simulink model "Prj1CDig_ZOH"  (R2026b)
settings: Solver=ode23s  StopTime=3600  RelTol=1e-8  EnableMultiTasking=on
undefined symbols (not defined in the file): Am, AmpW0, Bm, DiscIntNeverNeededParam, KI, KP, Kp, PO, Sat, Ta, Td, Tp1, Tp2, Ts, w0
settings Model: Creator=Adolfo  LastModifiedBy=Santana
settings SolverCC: MaxConsecutiveMinStep=5  ZeroCrossControl=DisableAll
settings DataIOCC: LimitDataPoints=on  MaxDataPoints=25000  ReturnWorkspaceOutputs=off  SaveFormat=Array  SignalLoggingSaveFormat=ModelDataLogs
settings OptimizationCC: BlockReduction=off  BooleanDataType=off  LifeSpan=inf  MemsetInitFltsAndDblsToZero=off  ReuseModelBlockBuffer=off
settings DebuggingCC: ArithmeticOperatorsInVariantConditions=warning  FcnCallInpInsideContextMsg=warning  MergeDetectMultiDrivingBlocksExec=none  MultiTaskCondExecSysMsg=none  MultiTaskDSMMsg=warning  SFExecutionAtInitializationDiag=none  SFNoUnconditionalDefaultTransitionDiag=warning  SFUnexpectedBacktrackingDiag=warning  SaveWithParameterizedLinksMsg=none  SignalResolutionControl=TryResolveAllWithWarning  StateNameClashWarn=warning  UnderspecifiedInitializationDetection=Classic
settings HardwareCC: ProdEndianess=Unspecified  ProdHWDeviceType=32-bit Generic  ProdIntDivRoundTo=Undefined  ProdLargestAtomicFloat=None  TargetUnknown=on
settings ModelReferenceCC: PropagateSignalLabelsOutOfModel=off
settings SFSimCC: CustomCodeUndefinedFunction=UseInterfaceOnly  SimUseLocalCustomCode=off
settings RTWCC: RTWUseLocalCustomCode=off
settings CodeAppCC: StateflowObjectComments=on
settings GRTTargetCC: CombineOutputUpdateFcns=off  GRTInterface=on  TargetFcnLib=ansi_tfl_tmw.mat  TargetLangStandard=C89/C90 (ANSI)
settings ConfigComp: CovSaveCumulativeToWorkspaceVar=on  CovSaveSingleToWorkspaceVar=on

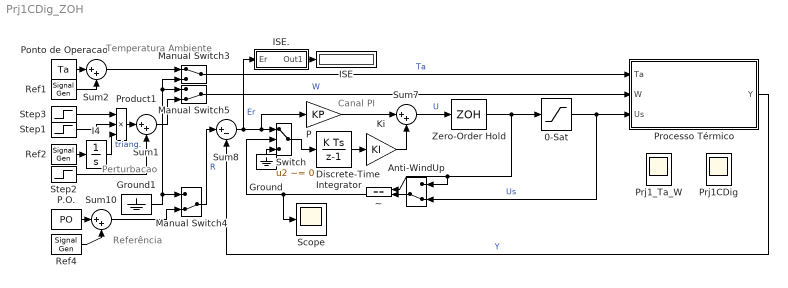
== system Prj1CDig_ZOH ==
  note: Referência
  note: Perturbacao
  note: Canal PI
  note: Temperatura Ambiente
  0-Sat : Saturate  UpperLimit=Sat  LowerLimit=0
  Anti-WindUp : ManualSwitch  CurrentSetting=0
  Discrete-Time Integrator : DiscreteIntegrator  SampleTime=Ts  ICPrevOutput=DiscIntNeverNeededParam  ICPrevScaledInput=DiscIntNeverNeededParam
  Ground : Ground
  Ground1 : Ground
  I4 : Integrator
  ISE : Display
  ISE. : Subsystem
  Ki : Gain  Gain=KI
  Manual Switch3 : ManualSwitch
  Manual Switch4 : ManualSwitch  CurrentSetting=0
  Manual Switch5 : ManualSwitch  CurrentSetting=0
  P : Gain  Gain=KP
  P.O. : Constant  Value=PO
  Ponto de Operacao : Constant  Value=Ta
  Prj1CDig : Scope
      settings: IsFloating=on  Floating=on  TimeSpan=3600  ActiveDisplayYMinimum=-200  ActiveDisplayYMaximum=1400  DataLoggingVariableName=ScopeData2
  Prj1_Ta_W : Scope
      settings: IsFloating=on  Floating=on  TimeSpan=3600  ActiveDisplayYMinimum=-25  ActiveDisplayYMaximum=35
  Processo Térmico : Subsystem
  Product1 : Product  Inputs=3  RndMeth=Zero
  Ref1 : SignalGenerator  Amplitude=2  Frequency=1/3600/24
  Ref2 : SignalGenerator  WaveForm=square  Amplitude=AmpW0  Frequency=w0  Units=rad/sec
  Ref4 : SignalGenerator  WaveForm=square  Amplitude=5  Frequency=.00125
  Scope : Scope
      settings: ActiveDisplayYMinimum=-0.125  ActiveDisplayYMaximum=1.125
  Step1 : Step  Time=3000  InitialValue=-20  FinalValue=0  SampleTime=0
  Step2 : Step  Time=1000  FinalValue=-20  SampleTime=0
  Step3 : Step  Time=1800  SampleTime=0
  Sum{1..2,7,10} (4 alike) : Sum  Inputs=|++
  Sum8 : Sum  Inputs=|+-
  Switch : Switch  Criteria=u2 ~= 0  Threshold=1  SaturateOnIntegerOverflow=off  InputSameDT=off
  Zero-Order Hold : ZeroOrderHold  SampleTime=Ts
  ~ : RelationalOperator  Operator===  OutDataTypeStr=boolean  InputSameDT=off
  wires:
  Sum8/1 -> P/1, Switch/1, ISE./1(Er)  "Er"
  P/1 -> Sum7/1
  Manual Switch5/1 -> Processo Térmico/2(W)  "W"
  Manual Switch3/1 -> Processo Térmico/1(Ta)  "Ta"
  Ground1/1 -> Manual Switch4/1, Manual Switch5/1, Manual Switch3/2
  Manual Switch4/1 -> Sum8/1  "R"
  Sum1/1 -> Manual Switch5/2
  Sum2/1 -> Manual Switch3/1
  Sum10/1 -> Manual Switch4/2
  Step2/1 -> Sum1/2
  Product1/1 -> Sum1/1
  Processo Térmico/1(Y) -> Sum8/2  "Y"
  Sum7/1 -> Zero-Order Hold/1  "U"
  Step1/1 -> Product1/2
  Step3/1 -> Product1/1
  Ref2/1 -> I4/1
  P.O./1 -> Sum10/1
  Ref4/1 -> Sum10/2
  ISE./1(Out1) -> ISE/1
  I4/1 -> Product1/3  "triang."
  Ki/1 -> Sum7/2
  0-Sat/1 -> Anti-WindUp/2, Processo Térmico/3(Us)  "Us"
  ~/1 -> Scope/1, Switch/2
  Anti-WindUp/1 -> ~/2
  Ground/1 -> Switch/3
  Discrete-Time Integrator/1 -> Ki/1
  Switch/1 -> Discrete-Time Integrator/1
  Ref1/1 -> Sum2/2
  Ponto de Operacao/1 -> Sum2/1
  Zero-Order Hold/1 -> 0-Sat/1, Anti-WindUp/1, ~/1

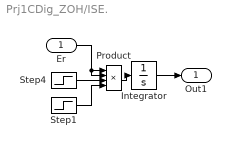
== system Prj1CDig_ZOH/ISE. ==
  Er : Inport
  Integrator : Integrator
  Product : Product  Inputs=4  RndMeth=Zero
  Step1 : Step  Time=3000  InitialValue=1  FinalValue=0  SampleTime=0
  Step4 : Step  Time=2100  SampleTime=0
  Out1 : Outport
  wires:
  Integrator/1 -> Out1/1
  Product/1 -> Integrator/1
  Step4/1 -> Product/3
  Er/1 -> Product/2, Product/1
  Step1/1 -> Product/4

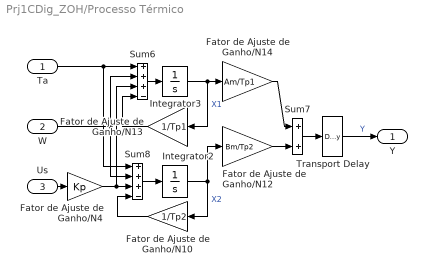
== system Prj1CDig_ZOH/Processo Térmico ==
  Ta : Inport
  W : Inport  Port=2
  Us : Inport  Port=3
  Fator de Ajuste de Ganho/N10 : Gain  Gain=1/Tp2  SaturateOnIntegerOverflow=on  OutDataTypeStr=Inherit: Same as input  ParamDataTypeStr=Inherit: Same as input
  Fator de Ajuste de Ganho/N12 : Gain  Gain=Bm/Tp2  SaturateOnIntegerOverflow=on  OutDataTypeStr=Inherit: Same as input  ParamDataTypeStr=Inherit: Same as input
  Fator de Ajuste de Ganho/N13 : Gain  Gain=1/Tp1  SaturateOnIntegerOverflow=on  OutDataTypeStr=Inherit: Same as input  ParamDataTypeStr=Inherit: Same as input
  Fator de Ajuste de Ganho/N14 : Gain  Gain=Am/Tp1  SaturateOnIntegerOverflow=on  OutDataTypeStr=Inherit: Same as input  ParamDataTypeStr=Inherit: Same as input
  Fator de Ajuste de Ganho/N4 : Gain  Gain=Kp  SaturateOnIntegerOverflow=on  OutDataTypeStr=Inherit: Same as input  ParamDataTypeStr=Inherit: Same as input
  Integrator2 : Integrator
  Integrator3 : Integrator
  Sum6 : Sum  Inputs=+++-
  Sum7 : Sum  InputSameDT=on  SaturateOnIntegerOverflow=on  OutDataTypeStr=Inherit: Same as first input
  Sum8 : Sum  Inputs=+++-
  Transport Delay : TransportDelay  DelayTime=Td  BufferSize=2048
  Y : Outport
  wires:
  Fator de Ajuste de Ganho/N12/1 -> Sum7/2
  Fator de Ajuste de Ganho/N13/1 -> Sum6/4
  Sum8/1 -> Integrator2/1
  Sum6/1 -> Integrator3/1
  Fator de Ajuste de Ganho/N10/1 -> Sum8/4
  Us/1 -> Fator de Ajuste de Ganho/N4/1
  Fator de Ajuste de Ganho/N14/1 -> Sum7/1
  Integrator3/1 -> Fator de Ajuste de Ganho/N14/1, Fator de Ajuste de Ganho/N13/1  "X1"
  Integrator2/1 -> Fator de Ajuste de Ganho/N12/1, Fator de Ajuste de Ganho/N10/1  "X2"
  Ta/1 -> Sum8/1, Sum6/1
  Fator de Ajuste de Ganho/N4/1 -> Sum6/3, Sum8/3
  Sum7/1 -> Transport Delay/1
  Transport Delay/1 -> Y/1  "Y"
  W/1 -> Sum6/2, Sum8/2
